simulink model "DKE"  (R2026b)
settings: Solver=ode4  StopTime=1000  FixedStep=1e-2
values from neighbouring files (symbols this model uses):
  a = R_e + h    (= 8000000)    [DKE_Parameters.m]    (also in disturbances_validation.m)
  A0 = eye(3)    [DKE_Parameters.m]    (also in disturbances_validation.m)
  A_body1_4 = 0.082716    [DKE_Parameters.m]    (also in disturbances_validation.m)
  A_body5_6 = 0.051076    [DKE_Parameters.m]    (also in disturbances_validation.m)
  A_panel = 0.0544    [DKE_Parameters.m]    (also in disturbances_validation.m)
  B1 = [+1; 0; 0]    [DKE_Parameters.m]    (also in disturbances_validation.m)
  B2 = [-1; 0; 0]    [DKE_Parameters.m]    (also in disturbances_validation.m)
  Bias_static = [1.8; -1.8; 1.8] * (1/3600) * (pi/180)    [DKE_Parameters.m]
  cos_FoV = cosd(FoV_half_deg)    [DKE_Parameters.m]
  e = 0.01    [DKE_Parameters.m]    (also in disturbances_validation.m = 0)
  epsilon = deg2rad(23.45)    [DKE_Parameters.m]    (also in disturbances_validation.m)
  f = 0.05    [DKE_Parameters.m]
  G = 6.67E-11    (= 6.67e-11)    [DKE_Parameters.m]    (also in disturbances_validation.m)
  H0 = sqrt(g10^2 + g11^2 + h11^2)    [DKE_Parameters.m]    (also in disturbances_validation.m)
  i = deg2rad(45)    [DKE_Parameters.m]    (also in disturbances_validation.m = deg2rad(0))
  I_depl = [Ixx, Ixy, Ixz ... (first row only)    [DKE_Parameters.m]    (also in disturbances_validation.m = diag([  Ix,   Iy,   Iz]))
  I_inv = I_depl \ eye(size(I_depl))    [DKE_Parameters.m]    (also in disturbances_validation.m = diag([1/Ix, 1/Iy, 1/Iz]))
  Ixx = 22.53E-2    (= 0.2253)    [DKE_Parameters.m]
  Iyy = 26.71E-2    (= 0.2671)    [DKE_Parameters.m]
  Izz = 33.03E-2    (= 0.3303)    [DKE_Parameters.m]
  j_B = [0.01; 0.05; 0.01]    [DKE_Parameters.m]    (also in disturbances_validation.m = [0 0 0])
  L1 = [0; 0; +1]    [DKE_Parameters.m]    (also in disturbances_validation.m)
  L2 = [0; +1; 0]    [DKE_Parameters.m]    (also in disturbances_validation.m)
  L3 = [0; 0; -1]    [DKE_Parameters.m]    (also in disturbances_validation.m)
  L4 = [0; -1; 0]    [DKE_Parameters.m]    (also in disturbances_validation.m)
  M_e = 5.97E24    (= 5.97e+24)    [DKE_Parameters.m]    (also in disturbances_validation.m)
  M_misalign = [1,  g_xy,  g_xz ... (first row only)    [DKE_Parameters.m]
  n_e = sqrt(mu_e/a^3)    [DKE_Parameters.m]
  n_s = 2*pi/T_s    (= 1.99102127766e-07)    [DKE_Parameters.m]    (also in disturbances_validation.m)
  omega = [0; 0; 0]    [disturbances_validation.m]
  omega_0 = [0.02; 0.05; 0.08]    [DKE_Parameters.m]
  omega_e = 2*pi/T_e    (= 7.29212351699e-05)    [DKE_Parameters.m]
  P = J_s/c    (= 4.52666666667e-06)    [DKE_Parameters.m]    (also in Panel_inertia_calc.m = 4.56e-06; disturbances_validation.m)
  Panel1 = [+1; 0; 0]    [DKE_Parameters.m]    (also in disturbances_validation.m)
  Panel2 = [+1; 0; 0]    [DKE_Parameters.m]    (also in disturbances_validation.m)
  Panel3 = [-1; 0; 0]    [DKE_Parameters.m]    (also in disturbances_validation.m)
  Panel4 = [-1; 0; 0]    [DKE_Parameters.m]    (also in disturbances_validation.m)
  r_CM = [0.015; 0.02; 0]    [DKE_Parameters.m]    (also in disturbances_validation.m = [0; 0; 0])
  R_e = 6371E3    (= 6371000)    [DKE_Parameters.m]
  r_s = 1.496E11    (= 149600000000)    [DKE_Parameters.m]
  rF1 = [0; 0; +0.113]    [DKE_Parameters.m]    (also in disturbances_validation.m)
  rF10 = [0; -0.273; 0]    [DKE_Parameters.m]    (also in disturbances_validation.m)
  rF2 = [0; +0.113; 0]    [DKE_Parameters.m]    (also in disturbances_validation.m)
  rF3 = [0; 0; -0.113]    [DKE_Parameters.m]    (also in disturbances_validation.m)
  rF4 = [0; -0.113; 0]    [DKE_Parameters.m]    (also in disturbances_validation.m)
  rF5 = [+0.183; 0; 0]    [DKE_Parameters.m]    (also in disturbances_validation.m)
  rF6 = [-0.183; 0; 0]    [DKE_Parameters.m]    (also in disturbances_validation.m)
  rF7 = [0; +0.273; 0]    [DKE_Parameters.m]    (also in disturbances_validation.m)
  rF8 = [0; -0.273; 0]    [DKE_Parameters.m]    (also in disturbances_validation.m)
  rF9 = [0; +0.273; 0]    [DKE_Parameters.m]    (also in disturbances_validation.m)
  rho_d = 0.1    [DKE_Parameters.m]    (also in disturbances_validation.m)
  rho_s_body = 0.5    [DKE_Parameters.m]    (also in disturbances_validation.m)
  rho_s_panel = 0.1    [DKE_Parameters.m]    (also in disturbances_validation.m)
  S_catalog = S_all    [DKE_Parameters.m]
  S_T = S_catalog'    [DKE_Parameters.m]
  S_tilde = A_e * S_catalog    [DKE_Parameters.m]
  Scale_factor = [500; -450; 300]    [DKE_Parameters.m]
  seed_u = randi(1000000, 1, N_stars)    [DKE_Parameters.m]
  seed_v = randi(1000000, 1, N_stars) + 1    [DKE_Parameters.m]
  theta_0 = deg2rad(100)    [DKE_Parameters.m]
  tilt_mag = deg2rad(11.5)    [DKE_Parameters.m]    (also in disturbances_validation.m = deg2rad(0))
  Ts = 0.01    [DKE_Parameters.m]
  var_uv = (f * tan(sigma_rad))^2    [DKE_Parameters.m]
undefined symbols (not defined in the file or in its folder): DiscIntNeverNeededParam
libraries: matrix_library x13, simulink x3
(part 1 of 2)
settings Model: Creator=romas  LastModifiedBy=annaa

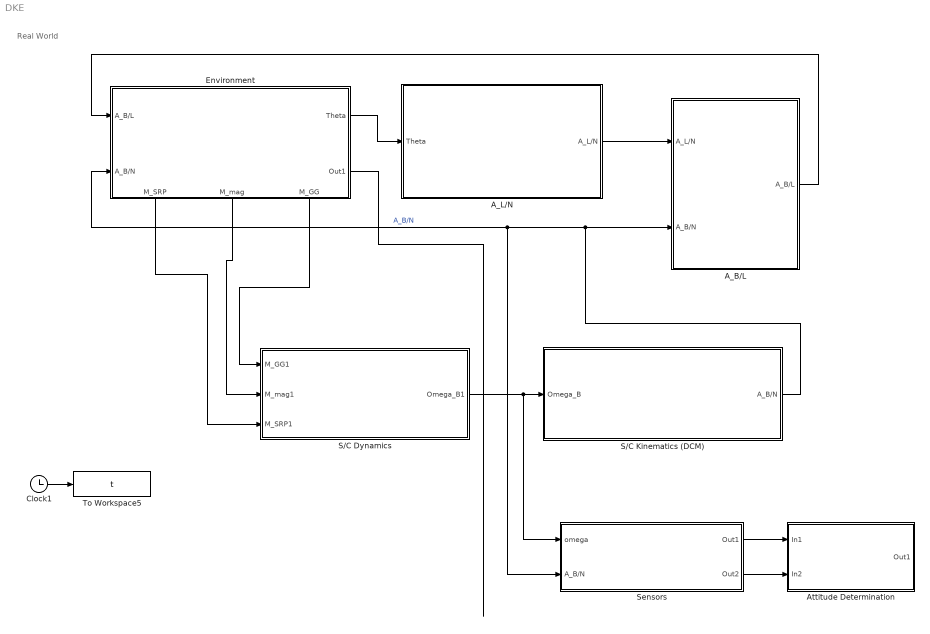
== system DKE ==
  note: Real World
  A_B/L : Subsystem
  A_L/N : Subsystem
  Attitude Determination : Subsystem
  Clock1 : Clock
  Environment : Subsystem
      settings: PortSchema="{\"entries\":[{\"content\":{\"sides\":[{\"content\":{\"connectorIds\":[\"In1\",\"In2\"]},\"type\":\"ConnectorPlacement.EquallySpacedRectSide\",\"uuid\":\"f27bd78b-7d48-4db2-bf8e-d3022e14d515\"},{\"content\":{\"connectorIds\":[\"Out1\",\"Out2\"],\"side\":\"RIGHT\"},\"type\":\"ConnectorPlacement.EquallySpacedRectSide\",\"uuid\":\"b376c0a4-a005-4a55-90c0-ee0846b30a39\"},{\"content\":{\"side\":\"TOP\"},\"type\":\"ConnectorPlacement.EquallySpacedRectSide\",\"uuid\":\"84036ad5-9f14-4563-9c1f-e71e951c9ec8\"},{\"content\":{\"connectorIds\":[\"Out3\",\"Out4\",\"Out5\"],\"side\":\"BOTTOM\"},\"type\":\"ConnectorPlacement.EquallySpacedRectSide\",\"uuid\":\"15031e61-cad9-40a6-8e15-8262f4115b8d\"}]},\"type\":\"ConnectorPlacement.EquallySpacedConnector\",\"uuid\":\"d1ace8d5-166e-4be1-ad70-b7223f3b1ea3\"}],\"packageUris\":[\"http://schema.mathworks.com/mf0/Connector/R2020b\"],\"version\":\"1.0\"}"
  S/C Dynamics : Subsystem
  S/C Kinematics (DCM) : Subsystem
  Sensors : Subsystem
  To Workspace5 : ToWorkspace  VariableName=t  SampleTime=-1
      settings: Save2DSignal=2-D array (concatenate along first dimension)
  wires:
  S/C Kinematics (DCM)/1(A_B/N) -> Sensors/2(A_B/N), Environment/2(A_B/N), A_B/L/2(A_B/N)  "A_B/N"
  Environment/1(Theta) -> A_L/N/1(Theta)
  S/C Dynamics/1(Omega_B1) -> Sensors/1(omega), S/C Kinematics (DCM)/1(Omega_B)
  Clock1/1 -> To Workspace5/1
  A_L/N/1(A_L/N) -> A_B/L/1(A_L/N)
  A_B/L/1(A_B/L) -> Environment/1(A_B/L)
  Environment/5(M_GG) -> S/C Dynamics/1(M_GG1)
  Environment/4(M_mag) -> S/C Dynamics/2(M_mag1)
  Environment/3(M_SRP) -> S/C Dynamics/3(M_SRP1)
  Environment/2(Out1) -> ?
  Sensors/1(Out1) -> Attitude Determination/1(In1)
  Sensors/2(Out2) -> Attitude Determination/2(In2)

== system DKE/A_B//L ==
  A_L/N : Inport
  A_B/N : Inport  Port=2
  MatrixMultiply1 : Product  Multiplication=Matrix(*)
  Transpose : Math  Operator=transpose
  A_B/L : Outport
  wires:
  A_B/N/1 -> MatrixMultiply1/2
  Transpose/1 -> MatrixMultiply1/1  "A_N/L"
  A_L/N/1 -> Transpose/1
  MatrixMultiply1/1 -> A_B/L/1  "A_B/L"

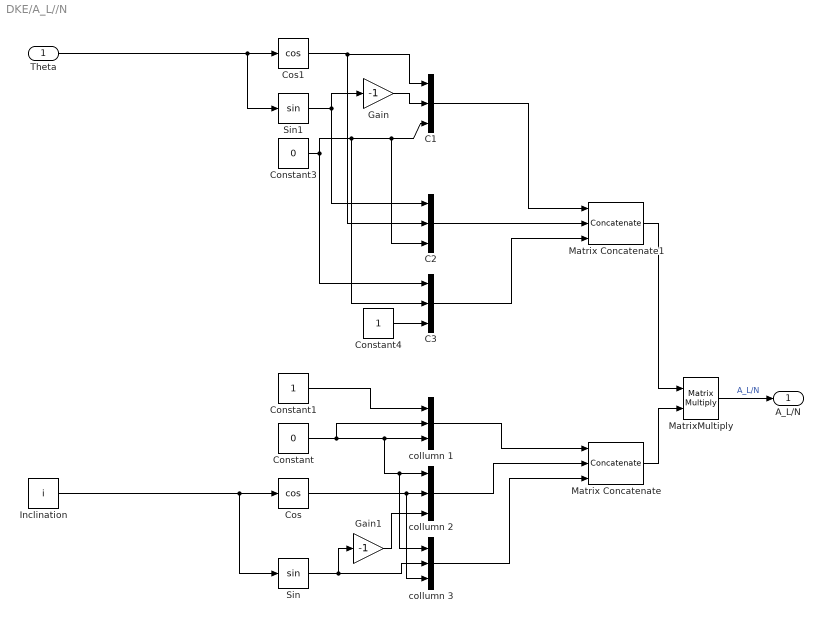
== system DKE/A_L//N ==
  Theta : Inport
  C1 : Mux  Inputs=3
  C2 : Mux  Inputs=3
  C3 : Mux  Inputs=3
  Constant : Constant  Value=0
  Constant1 : Constant
  Constant3 : Constant  Value=0
  Constant4 : Constant
  Cos : Trigonometry  Operator=cos
  Cos1 : Trigonometry  Operator=cos
  Gain : Gain  Gain=-1
  Gain1 : Gain  Gain=-1
  Inclination : Constant  Value=i
  Matrix Concatenate : Concatenate  NumInputs=3  Mode=Multidimensional array  ConcatenateDimension=2
  Matrix Concatenate1 : Concatenate  NumInputs=3  Mode=Multidimensional array  ConcatenateDimension=2
  MatrixMultiply : Product  Multiplication=Matrix(*)
  Sin : Trigonometry
  Sin1 : Trigonometry
  collumn 1 : Mux  Inputs=3
  collumn 2 : Mux  Inputs=3
  collumn 3 : Mux  Inputs=3
  A_L/N : Outport
  wires:
  collumn 3/1 -> Matrix Concatenate/3
  Inclination/1 -> Cos/1, Sin/1
  Sin/1 -> collumn 3/2, Gain1/1
  Theta/1 -> Sin1/1, Cos1/1
  Cos1/1 -> C1/1, C2/2
  Sin1/1 -> Gain/1, C2/1
  Gain/1 -> C1/2
  Constant3/1 -> C3/2, C2/3, C1/3, C3/1
  Constant4/1 -> C3/3
  Constant1/1 -> collumn 1/1
  Constant/1 -> collumn 1/2, collumn 3/1, collumn 2/1, collumn 1/3
  Cos/1 -> collumn 3/3, collumn 2/2
  Gain1/1 -> collumn 2/3
  collumn 1/1 -> Matrix Concatenate/1
  collumn 2/1 -> Matrix Concatenate/2
  C1/1 -> Matrix Concatenate1/1
  C2/1 -> Matrix Concatenate1/2
  C3/1 -> Matrix Concatenate1/3
  Matrix Concatenate1/1 -> MatrixMultiply/1
  Matrix Concatenate/1 -> MatrixMultiply/2
  MatrixMultiply/1 -> A_L/N/1  "A_L/N"

== system DKE/Attitude Determination ==
  note: ATTITUDE DETERINATION - Algebraic Method with pseudo-inverse
  In1 : Inport
  In2 : Inport  Port=2
  Constant3 : Constant  Value=S_catalog
  Constant5 : Constant  Value=S_T
  Display2 : Display
  Divide3 : Product  Inputs=*/  Multiplication=Matrix(*)
  Matrix Concatenate1 : Concatenate  NumInputs=3  Mode=Multidimensional array
  MatrixMultiply1 : Product  Multiplication=Matrix(*)
  Orthonormalization : Subsystem
  Product4 : Product
  Product5 : Product  Multiplication=Matrix(*)
  To Workspace3 : ToWorkspace  VariableName=A_est  SampleTime=-1
  Zero-Order Hold : ZeroOrderHold  SampleTime=0.2
  Out1 : Outport
  wires:
  Orthonormalization/1(Out1) -> Zero-Order Hold/1
  Constant5/1 -> Product5/2, MatrixMultiply1/2
  Matrix Concatenate1/1 -> Product4/1
  Product4/1 -> MatrixMultiply1/1  "S_w"
  In2/1 -> Matrix Concatenate1/3, Matrix Concatenate1/1, Matrix Concatenate1/2  "star_is_visible"
  Constant3/1 -> Product4/2
  MatrixMultiply1/1 -> Divide3/2  "M"
  In1/1 -> Product5/1  "O_w"
  Product5/1 -> Divide3/1  "B"
  Zero-Order Hold/1 -> Out1/1, To Workspace3/1, Display2/1  "A_est"
  Divide3/1 -> Orthonormalization/1(In1)  "A_B/N ST"

== system DKE/Environment ==
  A_B/L : Inport
  A_B/N : Inport  Port=2
  Constant : Constant  Value=[1;0;0]
  Constant1 : Constant  Value=[0; 0; 0]
  GG dynamics : Subsystem
  Magnetic torque : Subsystem
  MatrixMultiply : Product  Multiplication=Matrix(*)
  Orbital propagation : Subsystem
  SRP : Subsystem
  Switch : Switch  Criteria=u2 > Threshold  Threshold=0.5  SaturateOnIntegerOverflow=off  InputSameDT=off
  To Workspace1 : ToWorkspace  VariableName=M_mag  SampleTime=-1
      settings: Save2DSignal=2-D array (concatenate along first dimension)
  To Workspace2 : ToWorkspace  VariableName=M_srp  SampleTime=-1
      settings: Save2DSignal=2-D array (concatenate along first dimension)
  To Workspace3 : ToWorkspace  VariableName=M_gg  SampleTime=-1
      settings: Save2DSignal=2-D array (concatenate along first dimension)
  Theta : Outport
  Out1 : Outport  Port=2
  M_SRP : Outport  Port=3
  M_mag : Outport  Port=4
  M_GG : Outport  Port=5
  wires:
  Orbital propagation/4(r_hat) -> Magnetic torque/1(r_hat)
  A_B/N/1 -> Magnetic torque/2(A_B/N), Orbital propagation/1(A_B/N)
  Orbital propagation/1(Theta) -> Theta/1
  Magnetic torque/1(M_mag) -> To Workspace1/1, M_mag/1
  GG dynamics/1(M_GG) -> To Workspace3/1, M_GG/1
  Constant/1 -> MatrixMultiply/2
  MatrixMultiply/1 -> GG dynamics/1(C_Vector)  "C_Vector"
  A_B/L/1 -> MatrixMultiply/1
  Orbital propagation/3(S_Bhat) -> SRP/1(S_Bhat)
  Orbital propagation/5(r_Norm) -> GG dynamics/2(r_Norm), Magnetic torque/3(r_Norm)
  SRP/1(M_SRP) -> Switch/3
  Switch/1 -> M_SRP/1, To Workspace2/1
  Orbital propagation/2(Out1) -> Out1/1, Switch/2
  Constant1/1 -> Switch/1

== system DKE/S//C Dynamics ==
  note: $\text{Euler Equations - Constant Inertia Matrix} \\ \dot{\omega} = I^{-1} (\vec{T_{ext}} - \omega \times I\omega)$
  M_GG1 : Inport
  M_mag1 : Inport  Port=2
  M_SRP1 : Inport  Port=3
  Constant : Constant  Value=I_depl
  Constant1 : Constant  Value=I_inv
  Constant2 : Constant  Value=omega_0
  Cross Product : matrix_library/Cross Product
  Integrator : Integrator  InitialConditionSource=external  InitialCondition=omega
  Product : Product  Multiplication=Matrix(*)
  Product2 : Product  Multiplication=Matrix(*)
  Sum2 : Sum  Inputs=+++
  Sum3 : Sum  Inputs=+-
  Telemetry1 : Subsystem
  To Workspace : ToWorkspace  VariableName=omega_body  SampleTime=-1
  Omega_B1 : Outport
  wires:
  M_SRP1/1 -> Sum2/3
  M_mag1/1 -> Sum2/1
  M_GG1/1 -> Sum2/2
  Integrator/1 -> [omega_body], To Workspace/1, Omega_B1/1  "omega_body"
  Sum2/1 -> Sum3/1, Telemetry1/2(M_ext_total)  "M_ext_total"
  Cross Product/1 -> Sum3/2
  Product/1 -> Cross Product/2
  Constant/1 -> Product/1
  Sum3/1 -> Product2/2
  Constant1/1 -> Product2/1
  Product2/1 -> Integrator/1
  [omega_body] -> Telemetry1/1(Omega_B)
  [omega_body] -> Product/2, Cross Product/1
  Constant2/1 -> Integrator/2  "initial conditions for omega"

== system DKE/S//C Kinematics (DCM) ==
  note: $\text{Orthonormalization, Single Step}$
  Omega_B : Inport
  -[w] A_B/N : Product  Multiplication=Matrix(*)
  1/2AA^TA : Gain  Gain=1/2
  3/2A : Gain  Gain=3/2
  A A^T : Product  Multiplication=Matrix(*)
  AA^TA : Product  Multiplication=Matrix(*)
  Gain2 : Gain  Gain=-1
  Integrator : Integrator  InitialCondition=A0
  Sum : Sum  Inputs=+-
  Telemetry : Subsystem
  Transpose : Math  Operator=transpose
  skew matrix : Subsystem
  A_B/N : Outport
  wires:
  -[w] A_B/N/1 -> Integrator/1  "A_B/N_dot"
  Omega_B/1 -> skew matrix/1(w)
  Integrator/1 -> A A^T/1, 3/2A/1, Transpose/1, AA^TA/2  "A_B/N"
  AA^TA/1 -> 1/2AA^TA/1
  3/2A/1 -> Sum/1
  1/2AA^TA/1 -> Sum/2
  Sum/1 -> -[w] A_B/N/2, Telemetry/1(A_B/N), A_B/N/1  "3/2A -1/2AA^TA"
  skew matrix/1(omega_matrix) -> Gain2/1
  Transpose/1 -> A A^T/2
  A A^T/1 -> AA^TA/1
  Gain2/1 -> -[w] A_B/N/1

== system DKE/Sensors ==
  omega : Inport
  A_B/N : Inport  Port=2
  Gyro : Subsystem
  Star Tracker : Subsystem
  Out1 : Outport
  Out2 : Outport  Port=2
  wires:
  omega/1 -> Gyro/1(omega)
  A_B/N/1 -> Star Tracker/1(A_B/N)
  Star Tracker/1(Out1) -> Out1/1
  Star Tracker/2(Out2) -> Out2/1

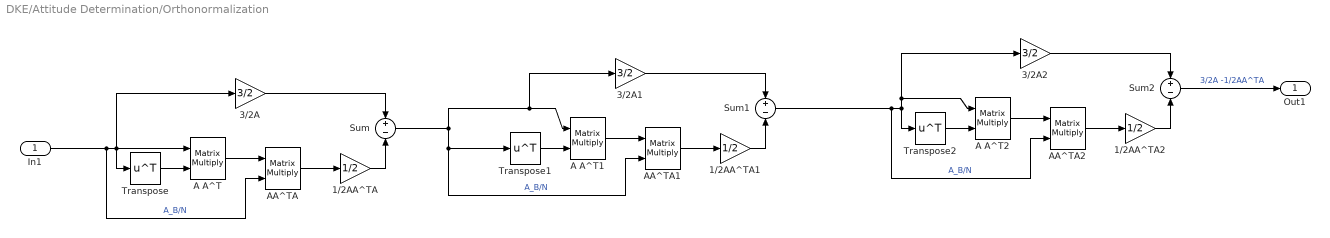
== system DKE/Attitude Determination/Orthonormalization ==
  In1 : Inport
  1/2AA^TA : Gain  Gain=1/2
  1/2AA^TA1 : Gain  Gain=1/2
  1/2AA^TA2 : Gain  Gain=1/2
  3/2A : Gain  Gain=3/2
  3/2A1 : Gain  Gain=3/2
  3/2A2 : Gain  Gain=3/2
  A A^T : Product  Multiplication=Matrix(*)
  A A^T1 : Product  Multiplication=Matrix(*)
  A A^T2 : Product  Multiplication=Matrix(*)
  AA^TA : Product  Multiplication=Matrix(*)
  AA^TA1 : Product  Multiplication=Matrix(*)
  AA^TA2 : Product  Multiplication=Matrix(*)
  Sum : Sum  Inputs=+-
  Sum1 : Sum  Inputs=+-
  Sum2 : Sum  Inputs=+-
  Transpose : Math  Operator=transpose
  Transpose1 : Math  Operator=transpose
  Transpose2 : Math  Operator=transpose
  Out1 : Outport
  wires:
  1/2AA^TA/1 -> Sum/2
  Transpose/1 -> A A^T/2
  AA^TA/1 -> 1/2AA^TA/1
  3/2A/1 -> Sum/1
  In1/1 -> A A^T/1, 3/2A/1, Transpose/1, AA^TA/2  "A_B/N"
  A A^T/1 -> AA^TA/1
  1/2AA^TA1/1 -> Sum1/2
  Transpose1/1 -> A A^T1/2
  AA^TA1/1 -> 1/2AA^TA1/1
  3/2A1/1 -> Sum1/1
  A A^T1/1 -> AA^TA1/1
  Sum2/1 -> Out1/1  "3/2A -1/2AA^TA"
  1/2AA^TA2/1 -> Sum2/2
  Transpose2/1 -> A A^T2/2
  AA^TA2/1 -> 1/2AA^TA2/1
  3/2A2/1 -> Sum2/1
  Sum1/1 -> A A^T2/1, 3/2A2/1, Transpose2/1, AA^TA2/2  "A_B/N"
  A A^T2/1 -> AA^TA2/1
  Sum/1 -> 3/2A1/1, A A^T1/1, AA^TA1/2, Transpose1/1  "A_B/N"

== system DKE/Environment/GG dynamics ==
  note: -(3GMt)/r^3
  C_Vector : Inport
  r_Norm : Inport  Port=2
  3GMt : Constant  Value=3*G*M_e
  Constant : Constant  Value=3
  Divide : Product  Inputs=*/
  Gain : Gain  Gain=-1
  Math Function : Math  Operator=pow
  Mux : Mux  Inputs=3
  Product{,1..5} (6 alike) : Product
  Subsystem : Subsystem
  c_vector_demux : Subsystem
  M_GG : Outport
  wires:
  Math Function/1 -> Divide/2
  3GMt/1 -> Divide/1
  Constant/1 -> Math Function/2
  Divide/1 -> Gain/1
  C_Vector/1 -> c_vector_demux/1(C_Vector)
  r_Norm/1 -> Math Function/1
  Gain/1 -> Product/2, Product4/2, Product2/2
  Subsystem/1(Kx) -> Product/1  "kx"
  c_vector_demux/1(c2c3) -> Product1/1  "c2c3"
  Product/1 -> Product1/2
  Product1/1 -> Mux/1
  Subsystem/2(Ky) -> Product2/1  "ky"
  c_vector_demux/2(c1c3) -> Product3/2  "c1c3"
  Product2/1 -> Product3/1
  Product3/1 -> Mux/2
  Subsystem/3(Kz) -> Product4/1  "kz"
  Product5/1 -> Mux/3
  Product4/1 -> Product5/2
  c_vector_demux/3(c2c1) -> Product5/1  "c2c1"
  Mux/1 -> M_GG/1

== system DKE/Environment/Magnetic torque ==
  r_hat : Inport
  A_B/N : Inport  Port=2
  r_Norm : Inport  Port=3
  Constant1 : Constant  Value=j_B
  Constant2 : Constant  Value=3
  Cross Product : matrix_library/Cross Product
  Divide : Product  Inputs=*/
  Dot Product : DotProduct  OutDataTypeStr=Inherit: Inherit via internal rule
  Gain : Gain  Gain=3
  Matrix Multiply : Product  Multiplication=Matrix(*)
  Power : Math  Operator=pow
  Product : Product
  Product1 : Product
  R_E^3 * H0 : Constant  Value=R_e^3*H0
  Sum : Sum  Inputs=|-+
  m_hat vector : Subsystem
  M_mag : Outport
  wires:
  Power/1 -> Divide/2
  r_Norm/1 -> Power/1
  Constant2/1 -> Power/2
  Cross Product/1 -> M_mag/1  "M_mag"
  Constant1/1 -> Cross Product/1
  Matrix Multiply/1 -> Cross Product/2  "b_B"
  A_B/N/1 -> Matrix Multiply/1
  Product1/1 -> Matrix Multiply/2  "b_N"
  Divide/1 -> Product1/2
  Sum/1 -> Product1/1
  R_E^3 * H0/1 -> Divide/1
  Product/1 -> Sum/2
  Gain/1 -> Product/1
  r_hat/1 -> Dot Product/2, Product/2  "r_hat"
  m_hat vector/1(m_hat) -> Dot Product/1, Sum/1  "m_hat"
  Dot Product/1 -> Gain/1  "dot(m_hat,r_hat)"

== system DKE/Environment/Orbital propagation ==
  A_B/N : Inport
  Eclipse : Subsystem
  Sun : Subsystem
  theta_dot : Subsystem
  Theta : Outport
  Out1 : Outport  Port=2
  S_Bhat : Outport  Port=3
  r_hat : Outport  Port=4
  r_Norm : Outport  Port=5
  wires:
  theta_dot/2(r_h) -> r_hat/1
  theta_dot/1(Theta) -> Theta/1
  A_B/N/1 -> theta_dot/1(A_B/N), Sun/1(A_B/N)
  Sun/1(S_Bhat) -> S_Bhat/1
  theta_dot/3(r_Norm) -> r_Norm/1
  Sun/2(Out1) -> Eclipse/1(In1)
  theta_dot/4(Out1) -> Eclipse/2(In2)
  Eclipse/1(Out1) -> Out1/1

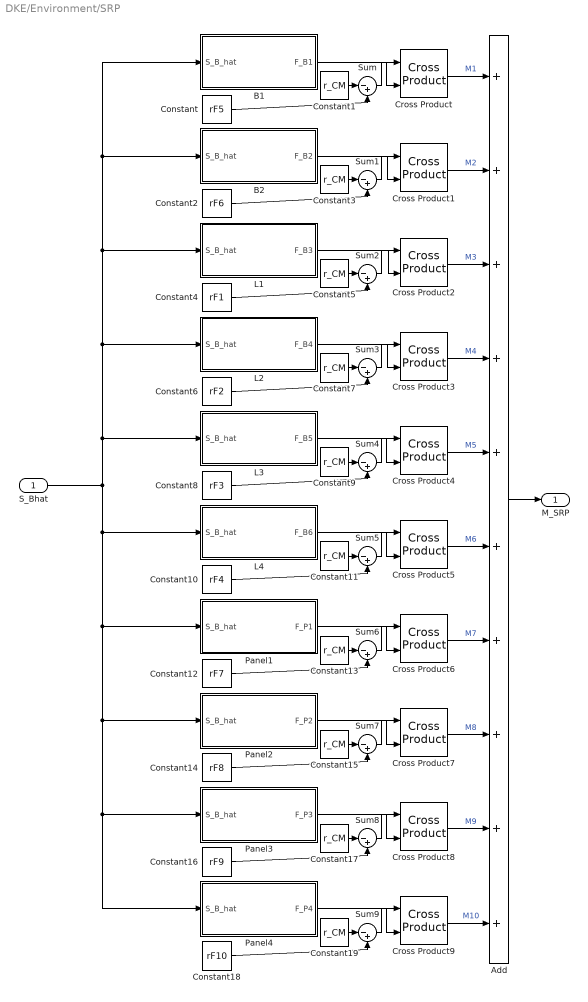
== system DKE/Environment/SRP ==
  S_Bhat : Inport
  Add : Sum  Inputs=++++++++++
  B1 : Subsystem
  B2 : Subsystem
  Constant : Constant  Value=rF5
  Constant{1,3,5,7,9,11,13,15,17,19} (10 alike) : Constant  Value=r_CM
  Constant10 : Constant  Value=rF4
  Constant12 : Constant  Value=rF7
  Constant14 : Constant  Value=rF8
  Constant16 : Constant  Value=rF9
  Constant18 : Constant  Value=rF10
  Constant2 : Constant  Value=rF6
  Constant4 : Constant  Value=rF1
  Constant6 : Constant  Value=rF2
  Constant8 : Constant  Value=rF3
  Cross Product{,1..9} (10 alike) : matrix_library/Cross Product
  L1 : Subsystem
  L2 : Subsystem
  L3 : Subsystem
  L4 : Subsystem
  Panel1 : Subsystem
  Panel2 : Subsystem
  Panel3 : Subsystem
  Panel4 : Subsystem
  Sum{,1..9} (10 alike) : Sum  Inputs=|-+
  M_SRP : Outport
  wires:
  Add/1 -> M_SRP/1
  Cross Product9/1 -> Add/10  "M10"
  Cross Product8/1 -> Add/9  "M9"
  Cross Product7/1 -> Add/8  "M8"
  Cross Product6/1 -> Add/7  "M7"
  Cross Product5/1 -> Add/6  "M6"
  Cross Product4/1 -> Add/5  "M5"
  Cross Product3/1 -> Add/4  "M4"
  Cross Product2/1 -> Add/3  "M3"
  Cross Product1/1 -> Add/2  "M2"
  Cross Product/1 -> Add/1  "M1"
  Sum9/1 -> Cross Product9/1
  Panel4/1(F_P4) -> Cross Product9/2
  Sum8/1 -> Cross Product8/1
  Panel3/1(F_P3) -> Cross Product8/2
  Sum7/1 -> Cross Product7/1
  Panel2/1(F_P2) -> Cross Product7/2
  Sum6/1 -> Cross Product6/1
  Panel1/1(F_P1) -> Cross Product6/2
  Sum5/1 -> Cross Product5/1
  L4/1(F_B6) -> Cross Product5/2
  Sum/1 -> Cross Product/1
  B1/1(F_B1) -> Cross Product/2
  Sum4/1 -> Cross Product4/1
  L3/1(F_B5) -> Cross Product4/2
  L2/1(F_B4) -> Cross Product3/2
  Sum3/1 -> Cross Product3/1
  L1/1(F_B3) -> Cross Product2/2
  Sum2/1 -> Cross Product2/1
  B2/1(F_B2) -> Cross Product1/2
  Sum1/1 -> Cross Product1/1
  Constant19/1 -> Sum9/1
  Constant18/1 -> Sum9/2
  Constant17/1 -> Sum8/1
  Constant16/1 -> Sum8/2
  Constant15/1 -> Sum7/1
  Constant14/1 -> Sum7/2
  Constant13/1 -> Sum6/1
  Constant12/1 -> Sum6/2
  Constant11/1 -> Sum5/1
  Constant10/1 -> Sum5/2
  Constant9/1 -> Sum4/1
  Constant8/1 -> Sum4/2
  Constant7/1 -> Sum3/1
  Constant6/1 -> Sum3/2
  Constant5/1 -> Sum2/1
  Constant4/1 -> Sum2/2
  Constant3/1 -> Sum1/1
  Constant2/1 -> Sum1/2
  Constant1/1 -> Sum/1
  Constant/1 -> Sum/2
  S_Bhat/1 -> L4/1(S_B_hat), Panel1/1(S_B_hat), Panel2/1(S_B_hat), Panel3/1(S_B_hat), Panel4/1(S_B_hat), L3/1(S_B_hat), L2/1(S_B_hat), L1/1(S_B_hat), B2/1(S_B_hat), B1/1(S_B_hat)

== system DKE/S//C Dynamics/Telemetry1 ==
  note: $\text{Checks for Dynamic Subsystem Correctness}$
  note: Moment Residual
  Omega_B : Inport
  M_ext_total : Inport  Port=2
  Constant : Constant  Value=I_depl
  Derivative : Derivative
  Display : Display
  Plot over Time : Scope
      settings: ActiveDisplayYMinimum=-5.1372521765431467E-5  ActiveDisplayYMaximum=0.00046762751742662116
  Product : Product  Multiplication=Matrix(*)
  Sum2 : Sum  Inputs=|-+
  norm : Subsystem
  wires:
  Sum2/1 -> norm/1(1)  "M - dH/dt = 0"
  Product/1 -> Derivative/1  "H"
  norm/1(Out1) -> Display/1, Plot over Time/1
  Omega_B/1 -> Product/2  "Omega"
  M_ext_total/1 -> Sum2/1
  Constant/1 -> Product/1
  Derivative/1 -> Sum2/2

== system DKE/S//C Kinematics (DCM)/Telemetry ==
  A_B/N : Inport
  AAT = 1 : Product  Multiplication=Matrix(*)
  Diagonal Check : Scope
      settings: ActiveDisplayYMinimum=0.99999999999995  ActiveDisplayYMaximum=1.00000000000005  DataLoggingVariableName=ScopeData2
  Extract Diagonal : matrix_library/Extract Diagonal
      settings: LibrarySourceBlock=|
      | simulink/Matrix
      | Operations/Extract Diagonal
  Last Iteration A : Display
  Last Iteration Residual off diagonal : Display
  Transpose1 : Math  Operator=transpose
  wires:
  A_B/N/1 -> Transpose1/1, AAT = 1/1, Last Iteration A/1
  Transpose1/1 -> AAT = 1/2
  AAT = 1/1 -> Extract Diagonal/1, Last Iteration Residual off diagonal/1
  Extract Diagonal/1 -> Diagonal Check/1

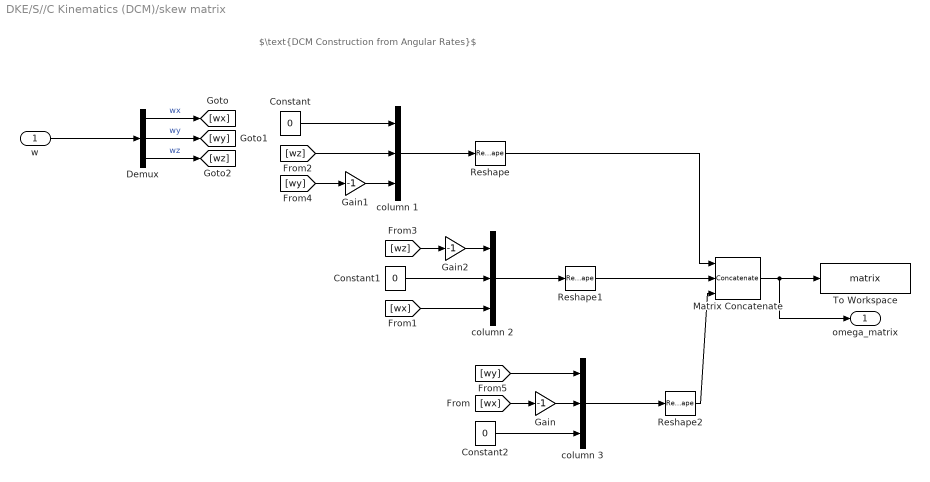
== system DKE/S//C Kinematics (DCM)/skew matrix ==
  note: $\text{DCM Construction from Angular Rates}$
  w : Inport
  Constant : Constant  Value=0
  Constant1 : Constant  Value=0
  Constant2 : Constant  Value=0
  Demux : Demux  Outputs=3
  Gain : Gain  Gain=-1
  Gain1 : Gain  Gain=-1
  Gain2 : Gain  Gain=-1
  Matrix Concatenate : Concatenate  NumInputs=3  Mode=Multidimensional array  ConcatenateDimension=2
  Reshape : Reshape  OutputDimensionality=Column vector (2-D)
  Reshape1 : Reshape  OutputDimensionality=Column vector (2-D)
  Reshape2 : Reshape  OutputDimensionality=Column vector (2-D)
  To Workspace : ToWorkspace  VariableName=matrix  SampleTime=-1
  column 1 : Mux  Inputs=3
  column 2 : Mux  Inputs=3
  column 3 : Mux  Inputs=3
  omega_matrix : Outport
  wires:
  Gain/1 -> column 3/2
  Gain1/1 -> column 1/3
  Constant/1 -> column 1/1
  Gain2/1 -> column 2/1
  Matrix Concatenate/1 -> To Workspace/1, omega_matrix/1
  column 1/1 -> Reshape/1
  column 2/1 -> Reshape1/1
  column 3/1 -> Reshape2/1
  Reshape/1 -> Matrix Concatenate/1
  Reshape1/1 -> Matrix Concatenate/2
  Reshape2/1 -> Matrix Concatenate/3
  w/1 -> Demux/1
  Constant1/1 -> column 2/2
  Constant2/1 -> column 3/3
  Demux/1 -> [wx]  "wx"
  [wx] -> Gain/1
  [wx] -> column 2/3
  Demux/3 -> [wz]  "wz"
  [wz] -> column 1/2
  [wz] -> Gain2/1
  Demux/2 -> [wy]  "wy"
  [wy] -> Gain1/1
  [wy] -> column 3/1

== system DKE/Sensors/Gyro ==
  omega : Inport
  Display : Display
  Gain : Gain  Gain=180/pi
  Gyroscope : Subsystem
  Integrator : Integrator
  Scope : Scope  NumInputPorts=2
      settings: ActiveDisplayYMinimum=-0.00607589525  ActiveDisplayYMaximum=0.0058140972500000006
  Scope1 : Scope
      settings: ActiveDisplayYMinimum=-0.004344809437227053  ActiveDisplayYMaximum=0.0039028388290876471
  Scope2 : Scope
      settings: ActiveDisplayYMinimum=-4.2395030543025944  ActiveDisplayYMaximum=38.155527488723358  DataLoggingVariableName=ScopeData3
  Subtract : Sum  Inputs=+-
  To Workspace : ToWorkspace  VariableName=omega_measured  SampleTime=-1
      settings: Save2DSignal=2-D array (concatenate along first dimension)
  To Workspace1 : ToWorkspace  VariableName=omega_ideal  SampleTime=-1
      settings: Save2DSignal=2-D array (concatenate along first dimension)
  norm : Subsystem
  wires:
  Integrator/1 -> norm/1(1)
  norm/1(Out1) -> Gain/1
  Gyroscope/2(omega_ideal) -> Subtract/2, To Workspace1/1, Scope1/1, Scope/2
  Gyroscope/1(omega_measured) -> Scope/1, Subtract/1, To Workspace/1
  Subtract/1 -> Integrator/1
  omega/1 -> Gyroscope/1(omega)
  Gain/1 -> Display/1, Scope2/1

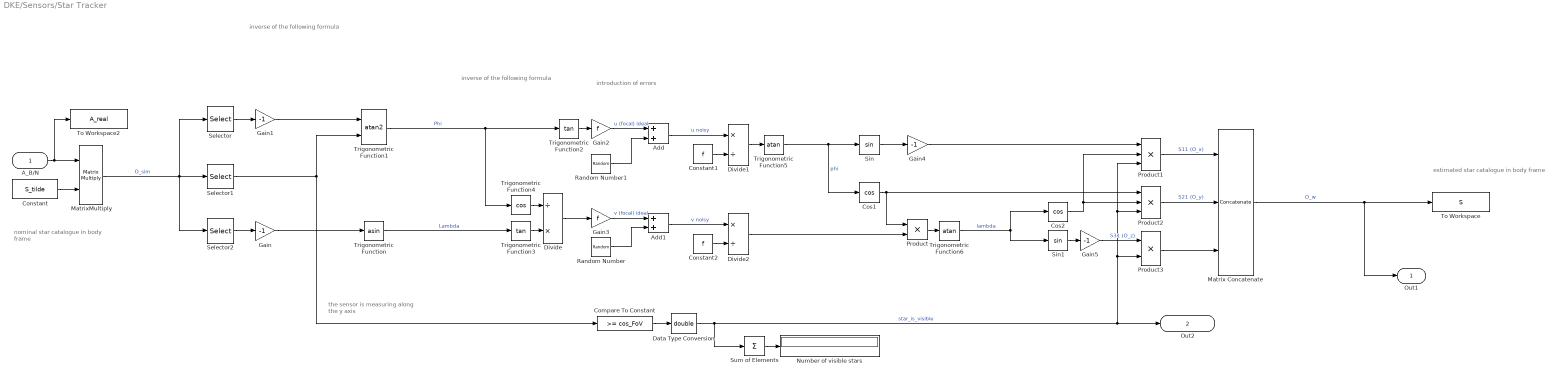
== system DKE/Sensors/Star Tracker ==
  note: estimated star catalogue in body frame
  note: nominal star catalogue in
      | body frame
  note: inverse of the following formula
  note: introduction of errors
  note: inverse of the following formula
  note: the sensor is measuring
      | along the y axis
  A_B/N : Inport
  Add : Sum
  Add1 : Sum
  Compare To Constant : simulink/Logic and Bit Operations/Compare To Constant  relop=>=  const=cos_FoV  OutDataTypeStr=boolean
  Constant : Constant  Value=S_tilde
  Constant1 : Constant  Value=f
  Constant2 : Constant  Value=f
  Cos1 : Trigonometry  Operator=cos
  Cos2 : Trigonometry  Operator=cos
  Data Type Conversion : DataTypeConversion  OutDataTypeStr=double  SaturateOnIntegerOverflow=off  RndMeth=Floor
  Divide : Product  Inputs=/*
  Divide1 : Product  Inputs=*/
  Divide2 : Product  Inputs=*/
  Gain{,1,4..5} (4 alike) : Gain  Gain=-1
  Gain2 : Gain  Gain=f
  Gain3 : Gain  Gain=f
  Matrix Concatenate : Concatenate  NumInputs=3  Mode=Multidimensional array
  MatrixMultiply : Product  Multiplication=Matrix(*)
  Number of visible stars : Display
  Product : Product
  Product1 : Product  Inputs=3
  Product2 : Product  Inputs=3
  Product3 : Product
  Random Number : RandomNumber  Variance=var_uv  Seed=seed_v  SampleTime=0.2
  Random Number1 : RandomNumber  Variance=var_uv  Seed=seed_u  SampleTime=0.2
  Selector : Selector  NumberOfDimensions=2  InputPortWidth=3  IndexOptions=Index vector (dialog),Select all  Indices=1,1  OutputSizes=1,1  RuntimeRangeChecks=off
  Selector1 : Selector  NumberOfDimensions=2  InputPortWidth=3  IndexOptions=Index vector (dialog),Select all  Indices=2,1  OutputSizes=1,1  RuntimeRangeChecks=off
  Selector2 : Selector  NumberOfDimensions=2  InputPortWidth=3  IndexOptions=Index vector (dialog),Select all  Indices=3,1  OutputSizes=1,1  RuntimeRangeChecks=off
  Sin : Trigonometry
  Sin1 : Trigonometry
  Sum of Elements : Sum  Inputs=+
  To Workspace : ToWorkspace  VariableName=S  SampleTime=-1
      settings: Save2DSignal=2-D array (concatenate along first dimension)
  To Workspace2 : ToWorkspace  VariableName=A_real  SampleTime=0.2
  Trigonometric Function : Trigonometry  Operator=asin
  Trigonometric Function1 : Trigonometry  Operator=atan2
  Trigonometric Function2 : Trigonometry  Operator=tan
  Trigonometric Function3 : Trigonometry  Operator=tan
  Trigonometric Function4 : Trigonometry  Operator=cos
  Trigonometric Function5 : Trigonometry  Operator=atan
  Trigonometric Function6 : Trigonometry  Operator=atan
  Out1 : Outport
  Out2 : Outport  Port=2
  wires:
  Constant/1 -> MatrixMultiply/2
  MatrixMultiply/1 -> Selector/1, Selector1/1, Selector2/1  "O_sim"
  Selector2/1 -> Gain/1
  Gain/1 -> Trigonometric Function/1
  Selector/1 -> Gain1/1
  Gain1/1 -> Trigonometric Function1/1
  Trigonometric Function1/1 -> Trigonometric Function2/1, Trigonometric Function4/1  "Phi"
  Trigonometric Function2/1 -> Gain2/1
  Gain2/1 -> Add/1  "u (focal) ideal"
  Trigonometric Function/1 -> Trigonometric Function3/1  "Lambda"
  Trigonometric Function4/1 -> Divide/1
  Divide/1 -> Gain3/1
  Gain3/1 -> Add1/1  "v (focal) ideal"
  Add/1 -> Divide1/1  "u noisy"
  Add1/1 -> Divide2/1  "v noisy"
  Constant1/1 -> Divide1/2
  Divide1/1 -> Trigonometric Function5/1
  Constant2/1 -> Divide2/2
  Divide2/1 -> Product/2
  Product/1 -> Trigonometric Function6/1
  Trigonometric Function5/1 -> Cos1/1, Sin/1  "phi"
  Sin/1 -> Gain4/1
  Gain4/1 -> Product1/1
  Trigonometric Function6/1 -> Cos2/1, Sin1/1  "lambda"
  Cos2/1 -> Product1/2, Product2/2
  Cos1/1 -> Product/1, Product2/1
  Product2/1 -> Matrix Concatenate/2  "S21 (O_y)"
  Sin1/1 -> Gain5/1
  Product1/1 -> Matrix Concatenate/1  "S11 (O_x)"
  Matrix Concatenate/1 -> Out1/1, To Workspace/1  "O_w"
  Gain5/1 -> Product3/1  "S31 (O_z)"
  Product3/1 -> Matrix Concatenate/3
  Selector1/1 -> Trigonometric Function1/2, Compare To Constant/1
  Compare To Constant/1 -> Data Type Conversion/1
  Data Type Conversion/1 -> Sum of Elements/1, Product1/3, Product2/3, Product3/2, Out2/1  "star_is_visible"
  Sum of Elements/1 -> Number of visible stars/1
  A_B/N/1 -> To Workspace2/1, MatrixMultiply/1
  Random Number1/1 -> Add/2
  Random Number/1 -> Add1/2
  Trigonometric Function3/1 -> Divide/2

== system DKE/Environment/GG dynamics/Subsystem ==
  Constant : Constant  Value=Ixx
  Constant1 : Constant  Value=Iyy
  Constant2 : Constant  Value=Izz
  Sum : Sum  Inputs=|+-
  Sum1 : Sum  Inputs=|+-
  Sum2 : Sum  Inputs=|+-
  Kx : Outport
  Ky : Outport  Port=2
  Kz : Outport  Port=3
  wires:
  Sum/1 -> Kx/1
  Constant/1 -> Sum1/2, Sum2/1
  Constant1/1 -> Sum2/2, Sum/1
  Constant2/1 -> Sum/2, Sum1/1
  Sum1/1 -> Ky/1
  Sum2/1 -> Kz/1

== system DKE/Environment/GG dynamics/c_vector_demux ==
  C_Vector : Inport
  Demux : Demux  Outputs=3
  Product : Product
  Product2 : Product
  Product3 : Product
  c2c3 : Outport
  c1c3 : Outport  Port=2
  c2c1 : Outport  Port=3
  wires:
  Product3/1 -> c2c1/1  "c2c1"
  Product2/1 -> c1c3/1  "c1c3"
  Demux/2 -> Product3/1, Product/1  "c2"
  Demux/3 -> Product2/2, Product/2  "c3"
  Demux/1 -> Product3/2, Product2/1  "c1"
  C_Vector/1 -> Demux/1
  Product/1 -> c2c3/1  "c2c3"

== system DKE/Environment/Magnetic torque/m_hat vector ==
  Clock : Clock
  Cos : Trigonometry  Operator=cos
  Cos1 : Trigonometry  Operator=cos
  Earth magnetic tilt : Constant  Value=tilt_mag
  Gain : Gain  Gain=omega_e
  Mux : Mux  Inputs=3
  Product : Product
  Product1 : Product
  Sin : Trigonometry
  Sin1 : Trigonometry
  m_hat : Outport
  wires:
  Cos/1 -> Mux/3
  Gain/1 -> Sin1/1, Cos1/1  "omega_E(t)"
  Cos1/1 -> Product/2
  Earth magnetic tilt/1 -> Sin/1, Cos/1
  Sin1/1 -> Product1/2
  Mux/1 -> m_hat/1  "m_hat"
  Sin/1 -> Product1/1, Product/1
  Product/1 -> Mux/1
  Clock/1 -> Gain/1
  Product1/1 -> Mux/2

== system DKE/Environment/Orbital propagation/Eclipse ==
  In1 : Inport
  In2 : Inport  Port=2
  AND : Logic  IconShape=distinctive  AllPortsSameDT=off  OutDataTypeStr=boolean
  Dot Product : DotProduct  OutDataTypeStr=Inherit: Inherit via internal rule
  Dot Product1 : DotProduct  OutDataTypeStr=Inherit: Inherit via internal rule
  One : Constant  Value=0  OutDataTypeStr=Inherit: Inherit via back propagation
  One1 : Constant  OutDataTypeStr=Inherit: Inherit via back propagation
  Scope : Scope
      settings: ActiveDisplayYMinimum=-0.12499999999999997  ActiveDisplayYMaximum=1.125  DataLoggingVariableName=ScopeData3
  Sqrt : Sqrt
  Square : Math  Operator=square
  Subtract : Sum  Inputs=+-
  Switch : Switch  Criteria=u2 > Threshold  SaturateOnIntegerOverflow=off  InputSameDT=off
  Switch1 : Switch  Criteria=u2 > Threshold  Threshold=R_e  SaturateOnIntegerOverflow=off  InputSameDT=off
  To Workspace : ToWorkspace  VariableName=its_eclipse_time  SampleTime=-1
      settings: Save2DSignal=2-D array (concatenate along first dimension)
  Zero : Constant  OutDataTypeStr=Inherit: Inherit via back propagation
  Zero1 : Constant  Value=0  OutDataTypeStr=Inherit: Inherit via back propagation
  Out1 : Outport
  wires:
  In1/1 -> Dot Product/2  "S_Nhat"
  In2/1 -> Dot Product/1, Dot Product1/2, Dot Product1/1  "r_N"
  Dot Product/1 -> Square/1, Switch/2  "d"
  Square/1 -> Subtract/2
  Dot Product1/1 -> Subtract/1
  Subtract/1 -> Sqrt/1
  One/1 -> Switch/1
  One1/1 -> Switch1/3
  Zero/1 -> Switch/3
  Zero1/1 -> Switch1/1
  Sqrt/1 -> Switch1/2
  Switch/1 -> AND/1
  Switch1/1 -> AND/2
  AND/1 -> Out1/1, To Workspace/1, Scope/1  "its_eclipse_time"

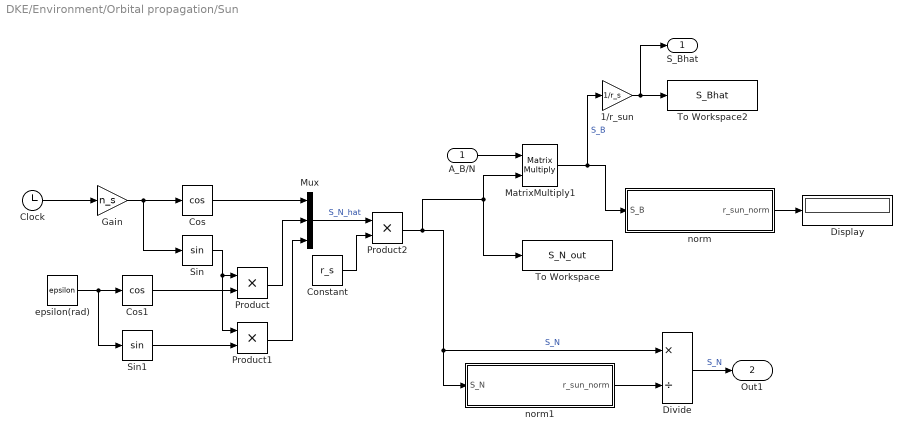
== system DKE/Environment/Orbital propagation/Sun ==
  A_B/N : Inport
  1/r_sun : Gain  Gain=1/r_s
  Clock : Clock
  Constant : Constant  Value=r_s
  Cos : Trigonometry  Operator=cos
  Cos1 : Trigonometry  Operator=cos
  Display : Display
  Divide : Product  Inputs=*/
  Gain : Gain  Gain=n_s
  MatrixMultiply1 : Product  Multiplication=Matrix(*)
  Mux : Mux  Inputs=3
  Product : Product
  Product1 : Product
  Product2 : Product
  Sin : Trigonometry
  Sin1 : Trigonometry
  To Workspace : ToWorkspace  VariableName=S_N_out  SampleTime=-1
      settings: Save2DSignal=2-D array (concatenate along first dimension)
  To Workspace2 : ToWorkspace  VariableName=S_Bhat  SaveFormat=Timeseries  SampleTime=-1
  epsilon(rad) : Constant  Value=epsilon
  norm : Subsystem
  norm1 : Subsystem
  S_Bhat : Outport
  Out1 : Outport  Port=2
  wires:
  Product2/1 -> Divide/1, norm1/1(S_N), To Workspace/1, MatrixMultiply1/2  "S_N"
  Constant/1 -> Product2/2
  Mux/1 -> Product2/1  "S_N_hat"
  Product1/1 -> Mux/3
  Sin1/1 -> Product1/2
  Product/1 -> Mux/2
  Cos1/1 -> Product/2
  Sin/1 -> Product/1, Product1/1
  epsilon(rad)/1 -> Cos1/1, Sin1/1
  Cos/1 -> Mux/1
  Gain/1 -> Cos/1, Sin/1
  Clock/1 -> Gain/1
  MatrixMultiply1/1 -> norm/1(S_B), 1/r_sun/1  "S_B"
  norm/1(r_sun_norm) -> Display/1
  1/r_sun/1 -> S_Bhat/1, To Workspace2/1
  A_B/N/1 -> MatrixMultiply1/1
  norm1/1(r_sun_norm) -> Divide/2
  Divide/1 -> Out1/1  "S_N"

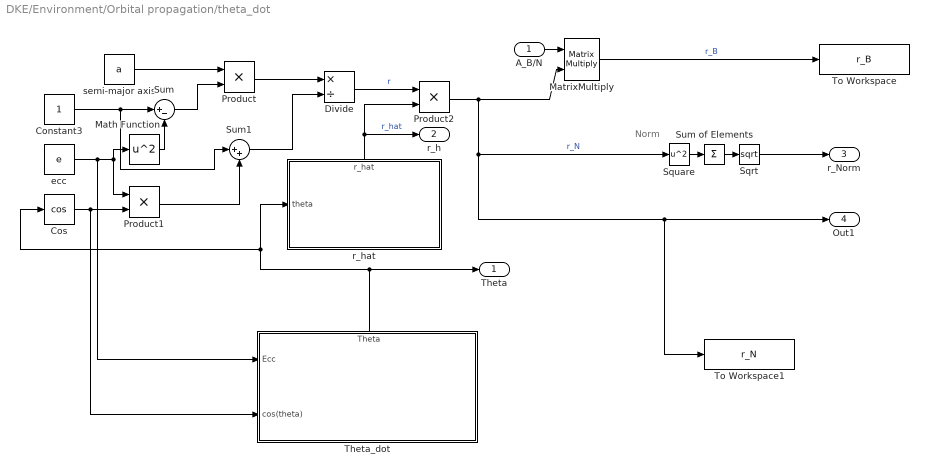
== system DKE/Environment/Orbital propagation/theta_dot ==
  note: Norm
  A_B/N : Inport
  Constant3 : Constant
  Cos : Trigonometry  Operator=cos
  Divide : Product  Inputs=*/
  Math Function : Math  Operator=square
  MatrixMultiply : Product  Multiplication=Matrix(*)
  Product : Product
  Product1 : Product
  Product2 : Product
  Sqrt : Sqrt
  Square : Math  Operator=square
  Sum : Sum  Inputs=|+-
  Sum of Elements : Sum  Inputs=+
  Sum1 : Sum  Inputs=|++
  Theta_dot : Subsystem
      settings: PortSchema="{\"entries\":[{\"content\":{\"sides\":[{\"content\":{\"connectorIds\":[\"In1\",\"In2\"]},\"type\":\"ConnectorPlacement.EquallySpacedRectSide\",\"uuid\":\"795c7f3f-5af3-4790-8464-7bc5e4ef34cb\"},{\"content\":{\"side\":\"RIGHT\"},\"type\":\"ConnectorPlacement.EquallySpacedRectSide\",\"uuid\":\"18aae6c2-ec45-4762-a70b-d706f89c58dd\"},{\"content\":{\"connectorIds\":[\"Out1\"],\"side\":\"TOP\"},\"type\":\"ConnectorPlacement.EquallySpacedRectSide\",\"uuid\":\"74038fb1-2674-4a5f-afa7-73cea69a66ba\"}]},\"type\":\"ConnectorPlacement.EquallySpacedConnector\",\"uuid\":\"03a5c504-3e80-4165-80c0-5738755afe64\"}],\"packageUris\":[\"http://schema.mathworks.com/mf0/Connector/R2020b\"],\"version\":\"1.0\"}"
  To Workspace : ToWorkspace  VariableName=r_B  SaveFormat=Timeseries  SampleTime=-1
  To Workspace1 : ToWorkspace  VariableName=r_N  SampleTime=-1
      settings: Save2DSignal=2-D array (concatenate along first dimension)
  ecc : Constant  Value=e
  r_hat : Subsystem
      settings: PortSchema="{\"entries\":[{\"content\":{\"sides\":[{\"content\":{\"connectorIds\":[\"In1\"]},\"type\":\"ConnectorPlacement.EquallySpacedRectSide\",\"uuid\":\"15aa9bf0-4304-4743-9146-86e71742f748\"},{\"content\":{\"side\":\"RIGHT\"},\"type\":\"ConnectorPlacement.EquallySpacedRectSide\",\"uuid\":\"3c2e279e-5a7b-45a5-8dfc-d1b79c479285\"},{\"content\":{\"connectorIds\":[\"Out1\"],\"side\":\"TOP\"},\"type\":\"ConnectorPlacement.EquallySpacedRectSide\",\"uuid\":\"c27605e1-4552-409d-9941-08da3bea576b\"}]},\"type\":\"ConnectorPlacement.EquallySpacedConnector\",\"uuid\":\"39bf02b2-a9a0-49e8-88d7-cfa6b47b7607\"}],\"packageUris\":[\"http://schema.mathworks.com/mf0/Connector/R2020b\"],\"version\":\"1.0\"}"
  semi-major axis : Constant  Value=a
  Theta : Outport
  r_h : Outport  Port=2
  r_Norm : Outport  Port=3
  Out1 : Outport  Port=4
  wires:
  Product2/1 -> Square/1, To Workspace1/1, Out1/1, MatrixMultiply/2  "r_N"
  Divide/1 -> Product2/1  "r"
  Sum1/1 -> Divide/2
  Product1/1 -> Sum1/2
  Cos/1 -> Theta_dot/2(cos(theta)), Product1/2
  ecc/1 -> Theta_dot/1(Ecc), Product1/1, Math Function/1
  Product/1 -> Divide/1
  Sum/1 -> Product/2
  Math Function/1 -> Sum/2
  Constant3/1 -> Sum1/1, Sum/1
  semi-major axis/1 -> Product/1
  MatrixMultiply/1 -> To Workspace/1  "r_B"
  A_B/N/1 -> MatrixMultiply/1
  Sqrt/1 -> r_Norm/1
  Theta_dot/1(Theta) -> Theta/1, r_hat/1(theta), Cos/1
  r_hat/1(r_hat) -> Product2/2, r_h/1  "r_hat"
  Square/1 -> Sum of Elements/1
  Sum of Elements/1 -> Sqrt/1

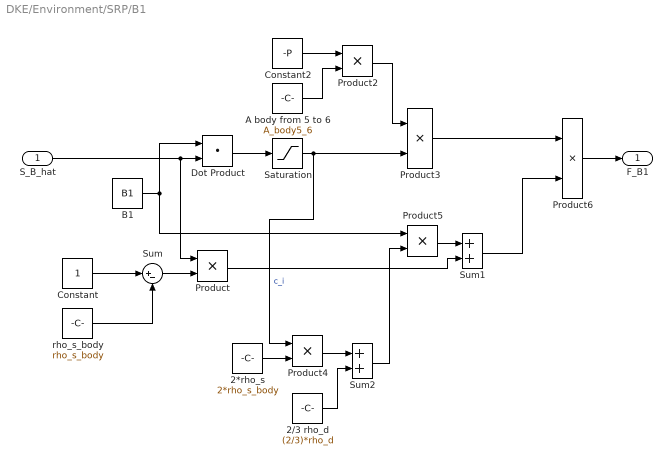
== system DKE/Environment/SRP/B1 ==
  S_B_hat : Inport
  2*rho_s : Constant  Value=2*rho_s_body
  2/3 rho_d : Constant  Value=(2/3)*rho_d
  A body from 5 to 6 : Constant  Value=A_body5_6
  B1 : Constant  Value=B1
  Constant : Constant
  Constant2 : Constant  Value=-P
  Dot Product : DotProduct  OutDataTypeStr=Inherit: Inherit via internal rule
  Product{,2..6} (6 alike) : Product
  Saturation : Saturate  UpperLimit=1  LowerLimit=0
  Sum : Sum  Inputs=|+-
  Sum1 : Sum
  Sum2 : Sum
  rho_s_body : Constant  Value=rho_s_body
  F_B1 : Outport
  wires:
  Constant2/1 -> Product2/1
  A body from 5 to 6/1 -> Product2/2
  Sum2/1 -> Product5/2
  Product/1 -> Sum1/2
  Constant/1 -> Sum/1
  Dot Product/1 -> Saturation/1
  B1/1 -> Dot Product/1, Product5/1
  2/3 rho_d/1 -> Sum2/2
  Sum/1 -> Product/2
  Saturation/1 -> Product4/1, Product3/2  "c_i"
  Product2/1 -> Product3/1
  Product3/1 -> Product6/1
  Product4/1 -> Sum2/1
  2*rho_s/1 -> Product4/2
  Sum1/1 -> Product6/2
  S_B_hat/1 -> Dot Product/2, Product/1
  rho_s_body/1 -> Sum/2
  Product6/1 -> F_B1/1
  Product5/1 -> Sum1/1

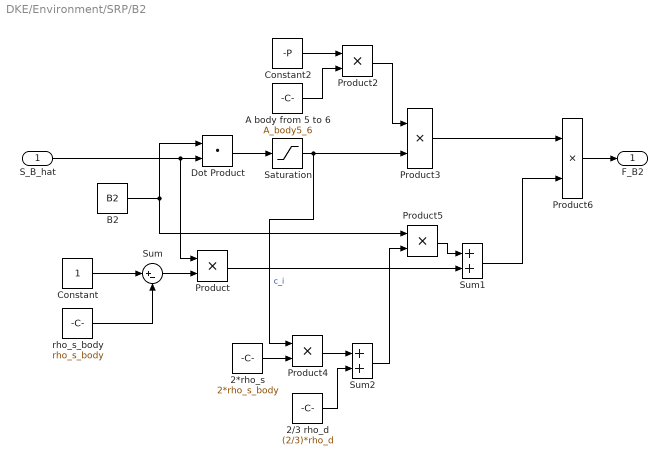
== system DKE/Environment/SRP/B2 ==
  S_B_hat : Inport
  2*rho_s : Constant  Value=2*rho_s_body
  2/3 rho_d : Constant  Value=(2/3)*rho_d
  A body from 5 to 6 : Constant  Value=A_body5_6
  B2 : Constant  Value=B2
  Constant : Constant
  Constant2 : Constant  Value=-P
  Dot Product : DotProduct  OutDataTypeStr=Inherit: Inherit via internal rule
  Product{,2..6} (6 alike) : Product
  Saturation : Saturate  UpperLimit=1  LowerLimit=0
  Sum : Sum  Inputs=|+-
  Sum1 : Sum
  Sum2 : Sum
  rho_s_body : Constant  Value=rho_s_body
  F_B2 : Outport
  wires:
  Product6/1 -> F_B2/1
  Constant2/1 -> Product2/1
  A body from 5 to 6/1 -> Product2/2
  Sum2/1 -> Product5/2
  Product/1 -> Sum1/2
  Constant/1 -> Sum/1
  Dot Product/1 -> Saturation/1
  B2/1 -> Dot Product/1, Product5/1
  2/3 rho_d/1 -> Sum2/2
  Sum/1 -> Product/2
  Saturation/1 -> Product4/1, Product3/2  "c_i"
  Product2/1 -> Product3/1
  Product3/1 -> Product6/1
  Product4/1 -> Sum2/1
  2*rho_s/1 -> Product4/2
  Sum1/1 -> Product6/2
  S_B_hat/1 -> Dot Product/2, Product/1
  rho_s_body/1 -> Sum/2
  Product5/1 -> Sum1/1

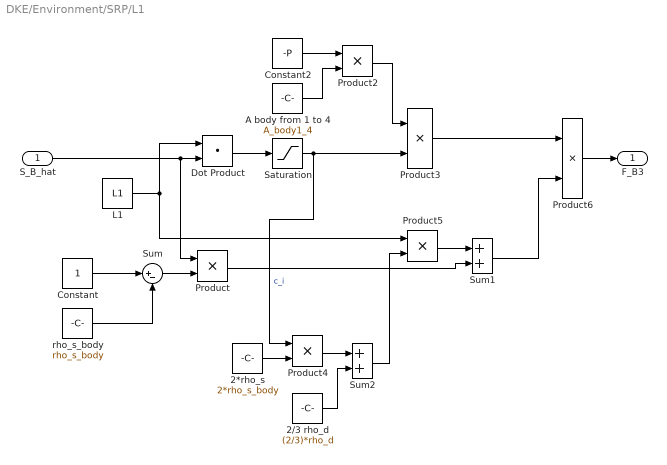
== system DKE/Environment/SRP/L1 ==
  S_B_hat : Inport
  2*rho_s : Constant  Value=2*rho_s_body
  2/3 rho_d : Constant  Value=(2/3)*rho_d
  A body from 1 to 4 : Constant  Value=A_body1_4
  Constant : Constant
  Constant2 : Constant  Value=-P
  Dot Product : DotProduct  OutDataTypeStr=Inherit: Inherit via internal rule
  L1 : Constant  Value=L1
  Product{,2..6} (6 alike) : Product
  Saturation : Saturate  UpperLimit=1  LowerLimit=0
  Sum : Sum  Inputs=|+-
  Sum1 : Sum
  Sum2 : Sum
  rho_s_body : Constant  Value=rho_s_body
  F_B3 : Outport
  wires:
  Product6/1 -> F_B3/1
  Constant2/1 -> Product2/1
  A body from 1 to 4/1 -> Product2/2
  Sum2/1 -> Product5/2
  Product/1 -> Sum1/2
  Constant/1 -> Sum/1
  Dot Product/1 -> Saturation/1
  L1/1 -> Dot Product/1, Product5/1
  2/3 rho_d/1 -> Sum2/2
  Sum/1 -> Product/2
  Saturation/1 -> Product4/1, Product3/2  "c_i"
  Product2/1 -> Product3/1
  Product3/1 -> Product6/1
  Product4/1 -> Sum2/1
  2*rho_s/1 -> Product4/2
  Sum1/1 -> Product6/2
  S_B_hat/1 -> Dot Product/2, Product/1
  rho_s_body/1 -> Sum/2
  Product5/1 -> Sum1/1

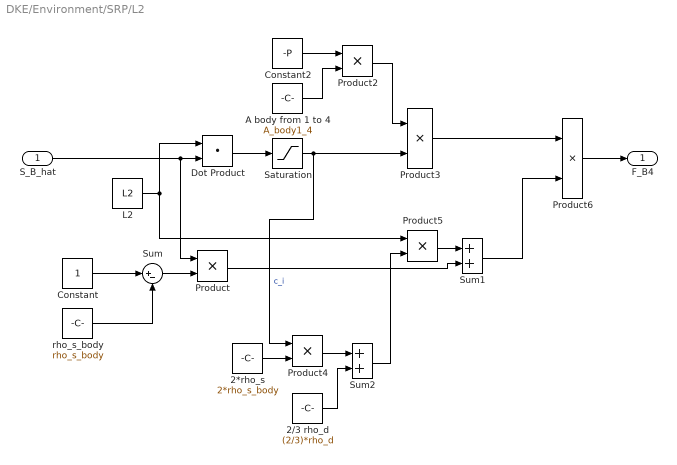
== system DKE/Environment/SRP/L2 ==
  S_B_hat : Inport
  2*rho_s : Constant  Value=2*rho_s_body
  2/3 rho_d : Constant  Value=(2/3)*rho_d
  A body from 1 to 4 : Constant  Value=A_body1_4
  Constant : Constant
  Constant2 : Constant  Value=-P
  Dot Product : DotProduct  OutDataTypeStr=Inherit: Inherit via internal rule
  L2 : Constant  Value=L2
  Product{,2..6} (6 alike) : Product
  Saturation : Saturate  UpperLimit=1  LowerLimit=0
  Sum : Sum  Inputs=|+-
  Sum1 : Sum
  Sum2 : Sum
  rho_s_body : Constant  Value=rho_s_body
  F_B4 : Outport
  wires:
  Product6/1 -> F_B4/1
  Constant2/1 -> Product2/1
  A body from 1 to 4/1 -> Product2/2
  Sum2/1 -> Product5/2
  Product/1 -> Sum1/2
  Constant/1 -> Sum/1
  Dot Product/1 -> Saturation/1
  L2/1 -> Dot Product/1, Product5/1
  2/3 rho_d/1 -> Sum2/2
  Sum/1 -> Product/2
  Saturation/1 -> Product4/1, Product3/2  "c_i"
  Product2/1 -> Product3/1
  Product3/1 -> Product6/1
  Product4/1 -> Sum2/1
  2*rho_s/1 -> Product4/2
  Sum1/1 -> Product6/2
  S_B_hat/1 -> Dot Product/2, Product/1
  rho_s_body/1 -> Sum/2
  Product5/1 -> Sum1/1

== system DKE/Environment/SRP/L3 ==
  S_B_hat : Inport
  2*rho_s : Constant  Value=2*rho_s_body
  2/3 rho_d : Constant  Value=(2/3)*rho_d
  A body from 1 to 4 : Constant  Value=A_body1_4
  Constant : Constant
  Constant2 : Constant  Value=-P
  Dot Product : DotProduct  OutDataTypeStr=Inherit: Inherit via internal rule
  L3 : Constant  Value=L3
  Product{,2..6} (6 alike) : Product
  Saturation : Saturate  UpperLimit=1  LowerLimit=0
  Sum : Sum  Inputs=|+-
  Sum1 : Sum
  Sum2 : Sum
  rho_s_body : Constant  Value=rho_s_body
  F_B5 : Outport
  wires:
  Constant2/1 -> Product2/1
  A body from 1 to 4/1 -> Product2/2
  Sum2/1 -> Product5/2
  Product/1 -> Sum1/2
  Constant/1 -> Sum/1
  Dot Product/1 -> Saturation/1
  L3/1 -> Dot Product/1, Product5/1
  2/3 rho_d/1 -> Sum2/2
  Sum/1 -> Product/2
  Saturation/1 -> Product4/1, Product3/2  "c_i"
  Product2/1 -> Product3/1
  Product3/1 -> Product6/1
  Product4/1 -> Sum2/1
  2*rho_s/1 -> Product4/2
  Sum1/1 -> Product6/2
  S_B_hat/1 -> Dot Product/2, Product/1
  rho_s_body/1 -> Sum/2
  Product6/1 -> F_B5/1
  Product5/1 -> Sum1/1

== system DKE/Environment/SRP/L4 ==
  S_B_hat : Inport
  2*rho_s : Constant  Value=2*rho_s_body
  2/3 rho_d : Constant  Value=(2/3)*rho_d
  A body from 1 to 4 : Constant  Value=A_body1_4
  Constant : Constant
  Constant2 : Constant  Value=-P
  Dot Product : DotProduct  OutDataTypeStr=Inherit: Inherit via internal rule
  L4 : Constant  Value=L4
  Product{,2..6} (6 alike) : Product
  Saturation : Saturate  UpperLimit=1  LowerLimit=0
  Sum : Sum  Inputs=|+-
  Sum1 : Sum
  Sum2 : Sum
  rho_s_body : Constant  Value=rho_s_body
  F_B6 : Outport
  wires:
  Constant2/1 -> Product2/1
  A body from 1 to 4/1 -> Product2/2
  Sum2/1 -> Product5/2
  Product/1 -> Sum1/2
  Constant/1 -> Sum/1
  Dot Product/1 -> Saturation/1
  L4/1 -> Dot Product/1, Product5/1
  2/3 rho_d/1 -> Sum2/2
  Sum/1 -> Product/2
  Saturation/1 -> Product4/1, Product3/2  "c_i"
  Product2/1 -> Product3/1
  Product3/1 -> Product6/1
  Product4/1 -> Sum2/1
  2*rho_s/1 -> Product4/2
  Sum1/1 -> Product6/2
  S_B_hat/1 -> Dot Product/2, Product/1
  rho_s_body/1 -> Sum/2
  Product6/1 -> F_B6/1
  Product5/1 -> Sum1/1

== system DKE/Environment/SRP/Panel1 ==
  S_B_hat : Inport
  2*rho_s : Constant  Value=2*rho_s_panel
  2/3 rho_d : Constant  Value=(2/3)*rho_d
  A_panel : Constant  Value=A_panel
  Constant : Constant
  Constant2 : Constant  Value=-P
  Dot Product : DotProduct  OutDataTypeStr=Inherit: Inherit via internal rule
  Panel1 : Constant  Value=Panel1
  Product{,2..6} (6 alike) : Product
  Saturation : Saturate  UpperLimit=1  LowerLimit=0
  Sum : Sum  Inputs=|+-
  Sum1 : Sum
  Sum2 : Sum
  rho_s_panel : Constant  Value=rho_s_panel
  F_P1 : Outport
  wires:
  Constant2/1 -> Product2/1
  A_panel/1 -> Product2/2
  Sum2/1 -> Product5/2
  Product/1 -> Sum1/2
  Constant/1 -> Sum/1
  Dot Product/1 -> Saturation/1
  Panel1/1 -> Dot Product/1, Product5/1
  2/3 rho_d/1 -> Sum2/2
  Sum/1 -> Product/2
  Saturation/1 -> Product4/1, Product3/2  "c_i"
  Product2/1 -> Product3/1
  Product3/1 -> Product6/1
  Product4/1 -> Sum2/1
  2*rho_s/1 -> Product4/2
  Sum1/1 -> Product6/2
  S_B_hat/1 -> Dot Product/2, Product/1
  rho_s_panel/1 -> Sum/2
  Product6/1 -> F_P1/1
  Product5/1 -> Sum1/1

== system DKE/Environment/SRP/Panel2 ==
  S_B_hat : Inport
  2*rho_s : Constant  Value=2*rho_s_panel
  2/3 rho_d : Constant  Value=(2/3)*rho_d
  A_panel : Constant  Value=A_panel
  Constant : Constant
  Constant2 : Constant  Value=-P
  Dot Product : DotProduct  OutDataTypeStr=Inherit: Inherit via internal rule
  Panel2 : Constant  Value=Panel2
  Product{,2..6} (6 alike) : Product
  Saturation : Saturate  UpperLimit=1  LowerLimit=0
  Sum : Sum  Inputs=|+-
  Sum1 : Sum
  Sum2 : Sum
  rho_s_panel : Constant  Value=rho_s_panel
  F_P2 : Outport
  wires:
  Constant2/1 -> Product2/1
  A_panel/1 -> Product2/2
  Sum2/1 -> Product5/2
  Product/1 -> Sum1/2
  Constant/1 -> Sum/1
  Dot Product/1 -> Saturation/1
  Panel2/1 -> Dot Product/1, Product5/1
  2/3 rho_d/1 -> Sum2/2
  Sum/1 -> Product/2
  Saturation/1 -> Product4/1, Product3/2  "c_i"
  Product2/1 -> Product3/1
  Product3/1 -> Product6/1
  Product4/1 -> Sum2/1
  2*rho_s/1 -> Product4/2
  Sum1/1 -> Product6/2
  S_B_hat/1 -> Dot Product/2, Product/1
  rho_s_panel/1 -> Sum/2
  Product6/1 -> F_P2/1
  Product5/1 -> Sum1/1

== system DKE/Environment/SRP/Panel3 ==
  S_B_hat : Inport
  2*rho_s : Constant  Value=2*rho_s_panel
  2/3 rho_d : Constant  Value=(2/3)*rho_d
  A_panel : Constant  Value=A_panel
  Constant : Constant
  Constant2 : Constant  Value=-P
  Dot Product : DotProduct  OutDataTypeStr=Inherit: Inherit via internal rule
  Panel3 : Constant  Value=Panel3
  Product{,2..6} (6 alike) : Product
  Saturation : Saturate  UpperLimit=1  LowerLimit=0
  Sum : Sum  Inputs=|+-
  Sum1 : Sum
  Sum2 : Sum
  rho_s_panel : Constant  Value=rho_s_panel
  F_P3 : Outport
  wires:
  Constant2/1 -> Product2/1
  A_panel/1 -> Product2/2
  Sum2/1 -> Product5/2
  Product/1 -> Sum1/2
  Constant/1 -> Sum/1
  Dot Product/1 -> Saturation/1
  Panel3/1 -> Dot Product/1, Product5/1
  2/3 rho_d/1 -> Sum2/2
  Sum/1 -> Product/2
  Saturation/1 -> Product4/1, Product3/2  "c_i"
  Product2/1 -> Product3/1
  Product3/1 -> Product6/1
  Product4/1 -> Sum2/1
  2*rho_s/1 -> Product4/2
  Sum1/1 -> Product6/2
  S_B_hat/1 -> Dot Product/2, Product/1
  rho_s_panel/1 -> Sum/2
  Product6/1 -> F_P3/1
  Product5/1 -> Sum1/1

== system DKE/Environment/SRP/Panel4 ==
  S_B_hat : Inport
  2*rho_s : Constant  Value=2*rho_s_panel
  2/3 rho_d : Constant  Value=(2/3)*rho_d
  A_panel : Constant  Value=A_panel
  Constant : Constant
  Constant2 : Constant  Value=-P
  Dot Product : DotProduct  OutDataTypeStr=Inherit: Inherit via internal rule
  Panel4 : Constant  Value=Panel4
  Product{,2..6} (6 alike) : Product
  Saturation : Saturate  UpperLimit=1  LowerLimit=0
  Sum : Sum  Inputs=|+-
  Sum1 : Sum
  Sum2 : Sum
  rho_s_panel : Constant  Value=rho_s_panel
  F_P4 : Outport
  wires:
  Constant2/1 -> Product2/1
  A_panel/1 -> Product2/2
  Sum2/1 -> Product5/2
  Product/1 -> Sum1/2
  Constant/1 -> Sum/1
  Dot Product/1 -> Saturation/1
  Panel4/1 -> Dot Product/1, Product5/1
  2/3 rho_d/1 -> Sum2/2
  Sum/1 -> Product/2
  Saturation/1 -> Product4/1, Product3/2  "c_i"
  Product2/1 -> Product3/1
  Product3/1 -> Product6/1
  Product4/1 -> Sum2/1
  2*rho_s/1 -> Product4/2
  Sum1/1 -> Product6/2
  S_B_hat/1 -> Dot Product/2, Product/1
  rho_s_panel/1 -> Sum/2
  Product6/1 -> F_P4/1
  Product5/1 -> Sum1/1

== system DKE/S//C Dynamics/Telemetry1/norm ==
  1 : Inport
  Sqrt : Sqrt
  Square : Math  Operator=square
  Sum of Elements : Sum  Inputs=+
  Out1 : Outport
  wires:
  Sqrt/1 -> Out1/1
  Sum of Elements/1 -> Sqrt/1
  Square/1 -> Sum of Elements/1
  1/1 -> Square/1

== system DKE/Sensors/Gyro/Gyroscope ==
  omega : Inport
  Band-Limited White Noise : simulink/Sources/Band-Limited White Noise  Cov=[1.218e-9; 1.218e-9; 1.218e-9]  Ts=Ts  seed=[23; 42; 101]
  Band-Limited White Noise1 : simulink/Sources/Band-Limited White Noise  Cov=[9.39e-14; 9.39e-14; 9.39e-14]  Ts=Ts  seed=[76; 1240; 3550]
  Bias_static : Constant  Value=Bias_static
  Constant : Constant  Value=M_misalign
  Discrete-Time Integrator1 : DiscreteIntegrator  SampleTime=-1  ICPrevOutput=DiscIntNeverNeededParam  ICPrevScaledInput=DiscIntNeverNeededParam
  MatrixMultiply1 : Product  Multiplication=Matrix(*)
  Quantizer : Quantizer  QuantizationInterval=8.7266e-5
  Saturation : Saturate  UpperLimit=2000  LowerLimit=-2000
  Scale_factor PPM : Gain  Gain=Scale_factor*1e-6
  Sum1 : Sum  Inputs=+++++
  Zero-Order Hold : ZeroOrderHold  SampleTime=-1
  omega_measured : Outport
  omega_ideal : Outport  Port=2
  wires:
  Zero-Order Hold/1 -> omega_measured/1
  Band-Limited White Noise/1 -> Sum1/3  "white noise"
  Band-Limited White Noise1/1 -> Discrete-Time Integrator1/1  "random walk"
  Scale_factor PPM/1 -> Sum1/2
  Sum1/1 -> Quantizer/1
  Quantizer/1 -> Saturation/1
  Saturation/1 -> Zero-Order Hold/1
  Bias_static/1 -> Sum1/1
  omega/1 -> omega_ideal/1, Scale_factor PPM/1, MatrixMultiply1/2
  Discrete-Time Integrator1/1 -> Sum1/4
  Constant/1 -> MatrixMultiply1/1
  MatrixMultiply1/1 -> Sum1/5

== system DKE/Sensors/Gyro/norm ==
  1 : Inport
  Sqrt : Sqrt
  Square : Math  Operator=square
  Sum of Elements : Sum  Inputs=+
  Out1 : Outport
  wires:
  Sqrt/1 -> Out1/1
  Sum of Elements/1 -> Sqrt/1
  Square/1 -> Sum of Elements/1
  1/1 -> Square/1

== system DKE/Environment/Orbital propagation/Sun/norm ==
  S_B : Inport
  Sqrt : Sqrt
  Square : Math  Operator=square
  Sum of Elements : Sum  Inputs=+
  r_sun_norm : Outport
  wires:
  Sqrt/1 -> r_sun_norm/1
  Sum of Elements/1 -> Sqrt/1
  Square/1 -> Sum of Elements/1
  S_B/1 -> Square/1

== system DKE/Environment/Orbital propagation/Sun/norm1 ==
  S_N : Inport
  Sqrt : Sqrt
  Square : Math  Operator=square
  Sum of Elements : Sum  Inputs=+
  r_sun_norm : Outport
  wires:
  S_N/1 -> Square/1
  Square/1 -> Sum of Elements/1
  Sum of Elements/1 -> Sqrt/1
  Sqrt/1 -> r_sun_norm/1
